simulink model "red_pitaya_adc"  (R2018a)
settings: Solver=VariableStepAuto  StartTime=0.0  StopTime=10.0  RelTol=1e-3
libraries: xbsIndex_r4 x5
settings Model: Creator=qwerty40  LastModifiedBy=hpw1
settings CodeAppCC: StateflowObjectComments=on

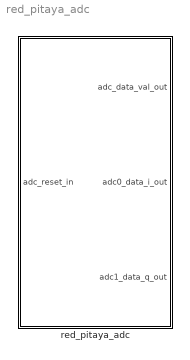
== system red_pitaya_adc ==
  red_pitaya_adc : Subsystem  Tag=xps:red_pitaya_adc  mask(adc){bits=14}
      mask prompts: bits "Number of bits:"
      mask help: Interface to ADC device available on Red Pitaya board
      mask init:
      | red_pitaya_adc_mask(gcb);
      mask TypeOptions bits: 10 | 14
      mask DialogControl Container6 Prompt: Parameters

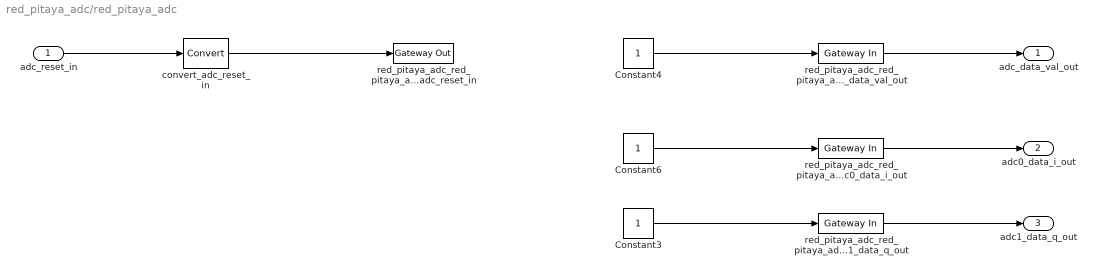
== system red_pitaya_adc/red_pitaya_adc ==
  adc_reset_in : Inport
  Constant3 : Constant
  Constant4 : Constant
  Constant6 : Constant
  convert_adc_reset_in : xbsIndex_r4/Convert  gui_display_data_type=Boolean  arith_type=Boolean  n_bits=16  bin_pt=14  float_type=Single  exp_bits=8  fraction_bits=24  quantization=Truncate  overflow=Wrap  en=off  latency=0  pipeline=off  dbl_ovrd=off  block_type=convert
  red_pitaya_adc_red_pitaya_adc_adc0_data_i_out : xbsIndex_r4/Gateway In  gui_display_data_type=Fixed-point  arith_type="Signed  (2's comp)"  n_bits=14  bin_pt=0  preci_type=Single  exp_width=8  frac_width=24  rows=1  columns=1  quantization=Truncate  overflow=Wrap  period=1  UseAsADC=off  ADCChannel='1'  interface=None  automatic_assignment=on  address_offset=hex2dec('00')  intf_name=''  intf_description=''  default_value=0  timing_constraint=None  locs_specified=off  LOCs={}  io_standard={}  inherit_from_input=off  hdl_port=on  dbl_ovrd=off  block_type=gatewayin
  red_pitaya_adc_red_pitaya_adc_adc1_data_q_out : xbsIndex_r4/Gateway In  gui_display_data_type=Fixed-point  arith_type="Signed  (2's comp)"  n_bits=14  bin_pt=0  preci_type=Single  exp_width=8  frac_width=24  rows=1  columns=1  quantization=Truncate  overflow=Wrap  period=1  UseAsADC=off  ADCChannel='1'  interface=None  automatic_assignment=on  address_offset=hex2dec('00')  intf_name=''  intf_description=''  default_value=0  timing_constraint=None  locs_specified=off  LOCs={}  io_standard={}  inherit_from_input=off  hdl_port=on  dbl_ovrd=off  block_type=gatewayin
  red_pitaya_adc_red_pitaya_adc_adc_data_val_out : xbsIndex_r4/Gateway In  gui_display_data_type=Boolean  arith_type=Boolean  n_bits=16  bin_pt=14  preci_type=Single  exp_width=8  frac_width=24  rows=1  columns=1  quantization="Round  (unbiased: +/- Inf)"  overflow=Saturate  period=1  UseAsADC=off  ADCChannel='1'  interface=None  automatic_assignment=on  address_offset=hex2dec('00')  intf_name=''  intf_description=''  default_value=0  timing_constraint=None  locs_specified=off  LOCs={}  io_standard={}  inherit_from_input=off  hdl_port=on  dbl_ovrd=off  block_type=gatewayin
  red_pitaya_adc_red_pitaya_adc_adc_reset_in : xbsIndex_r4/Gateway Out  inherit_from_input=off  hdl_port=on  rows=1  columns=1  UseAsDAC=off  DACChannel='1'  interface=None  automatic_assignment=on  address_offset=hex2dec('00')  intf_name=''  intf_description=''  timing_constraint=None  locs_specified=off  LOCs={}  io_standard={}  block_type=gatewayout
  adc_data_val_out : Outport
  adc0_data_i_out : Outport  Port=2
  adc1_data_q_out : Outport  Port=3
  wires:
  adc_reset_in/1 -> convert_adc_reset_in/1
  convert_adc_reset_in/1 -> red_pitaya_adc_red_pitaya_adc_adc_reset_in/1
  Constant4/1 -> red_pitaya_adc_red_pitaya_adc_adc_data_val_out/1
  Constant6/1 -> red_pitaya_adc_red_pitaya_adc_adc0_data_i_out/1
  Constant3/1 -> red_pitaya_adc_red_pitaya_adc_adc1_data_q_out/1
  red_pitaya_adc_red_pitaya_adc_adc_data_val_out/1 -> adc_data_val_out/1
  red_pitaya_adc_red_pitaya_adc_adc0_data_i_out/1 -> adc0_data_i_out/1
  red_pitaya_adc_red_pitaya_adc_adc1_data_q_out/1 -> adc1_data_q_out/1
